simulink model "AGV_Simulation_Follow"  (R2022a)
settings: Solver=VariableStepAuto  StartTime=0.0  StopTime=200  RelTol=1e-3  EnableMultiTasking=on
undefined symbols (not defined in the file or in its folder): Final_path, gray, lastx, lasty, Rec, SDTV, start
libraries: vrlib x6, visionconversions x2, robotalgslib x1, visionanalysis x1, visiontextngfix x1
settings Model: Creator=Carlos  LastModifiedBy=a22adhpa
settings SolverCC: AlgebraicLoopSolver=TrustRegion
settings DataIOCC: LimitDataPoints=on  MaxDataPoints=10000
settings OptimizationCC: LifeSpan=inf
settings DebuggingCC: UnconnectedInputMsg=warning  UnconnectedOutputMsg=warning  UnconnectedLineMsg=warning  AllowSymbolicDim=off  SFUnexpectedBacktrackingDiag=warning  SFNoUnconditionalDefaultTransitionDiag=warning  SFExecutionAtInitializationDiag=none  SFMachineParentedDataDiag=warning  UnderSpecifiedDimensionMsg=warning  ArithmeticOperatorsInVariantConditions=warning
settings SFSimCC: SimUseLocalCustomCode=off  CustomCodeUndefinedFunction=UseInterfaceOnly
settings RTWCC: RTWUseLocalCustomCode=off
settings CodeAppCC: StateflowObjectComments=on
settings GRTTargetCC: TargetLangStandard=C89/C90 (ANSI)
settings ConfigComp: CovMetricSettings=dw  CovSaveCumulativeToWorkspaceVar=on  CovSaveSingleToWorkspaceVar=on  CovExternalEMLEnable=off  CovSFcnEnable=off
settings SimscapeCC: SimscapeLogType=all  SimscapeLogSimulationStatistics=on  SimscapeLogDataHistory=10000

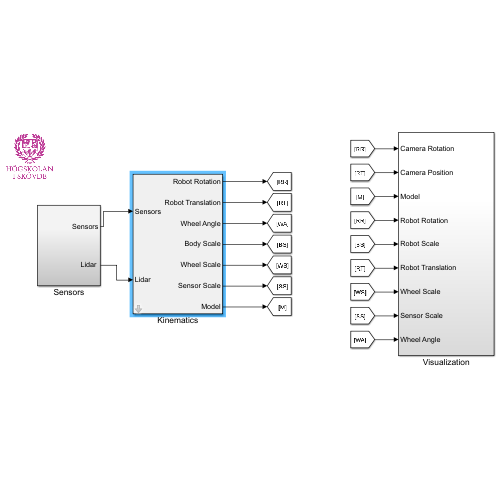
[thumbnail: Simulink's stored preview of the top-level diagram]
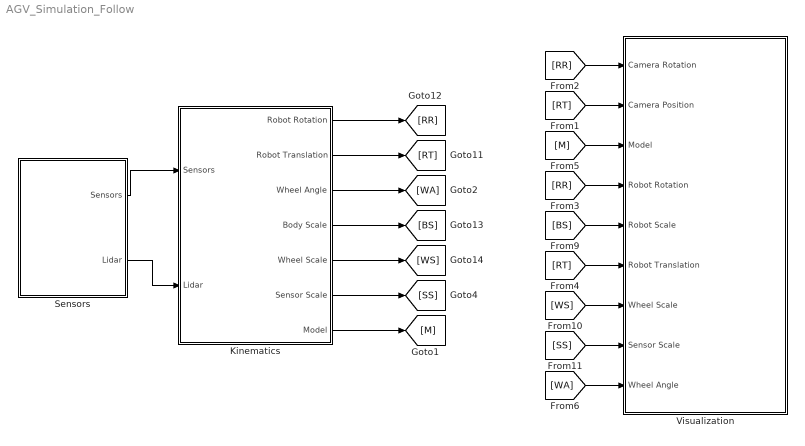
== system AGV_Simulation_Follow ==
  Kinematics : Subsystem  mask(Simulation Parameters){Op=Differential Drive, Kim=Inverse, DimR=[0.6, 0.5, 0.15], DimW=[0.18, 0.12], InitPos=start, InitRot=0, Dim=[1.00,1.00,0.15;1.40,0.80,0.15;1.40,0.8,0.15;1.2,0.8,0.15]}
      mask prompts: Op "Robot Models:"; Kim "Kinematics:"; DimR "Robot Dimensions (m)"; DimW "Wheel Dimensions (m)"; InitPos "Initial Position (m)"; InitRot "Initial Rotation (rad)"; Dim "Dimensions (m)"
      mask help: Define the dimensions of the robot [Length, Width, Thickness] and of the wheels [Radius, Thickness].
      mask TypeOptions Op: Differential Drive | Tricycle Drive | Ackermann Steering | Swedish Model
      mask TypeOptions Kim: Forward | Inverse
      mask DialogControl Control Prompt: Select the robot and kinematics used for the algorithms.
      mask DialogControl DescTextVar_copy Prompt: Define the dimensions of the robot [Length, Width, Thickness] and of the wheels [Radius, Thickness]:
      mask DialogControl DescTextVar Prompt: Set the initial position [X Z] and rotation [Angle] of the robot:
  Sensors : Subsystem
  Visualization : Subsystem
  wires:
  Kinematics/2(Robot Translation) -> [RT]
  Kinematics/1(Robot Rotation) -> [RR]
  Kinematics/4(Body Scale) -> [BS]
  Kinematics/5(Wheel Scale) -> [WS]
  Kinematics/6(Sensor Scale) -> [SS]
  Kinematics/7(Model) -> [M]
  [RR] -> Visualization/1(Camera Rotation)
  [RT] -> Visualization/2(Camera Position)
  [M] -> Visualization/3(Model)
  [RR] -> Visualization/4(Robot Rotation)
  [BS] -> Visualization/5(Robot Scale)
  [WS] -> Visualization/7(Wheel Scale)
  [SS] -> Visualization/8(Sensor Scale)
  Kinematics/3(Wheel Angle) -> [WA]
  [WA] -> Visualization/9(Wheel Angle)
  [RT] -> Visualization/6(Robot Translation)
  Sensors/1(Sensors) -> Kinematics/1(Sensors)
  Sensors/2("Lidar ") -> Kinematics/2(Lidar)

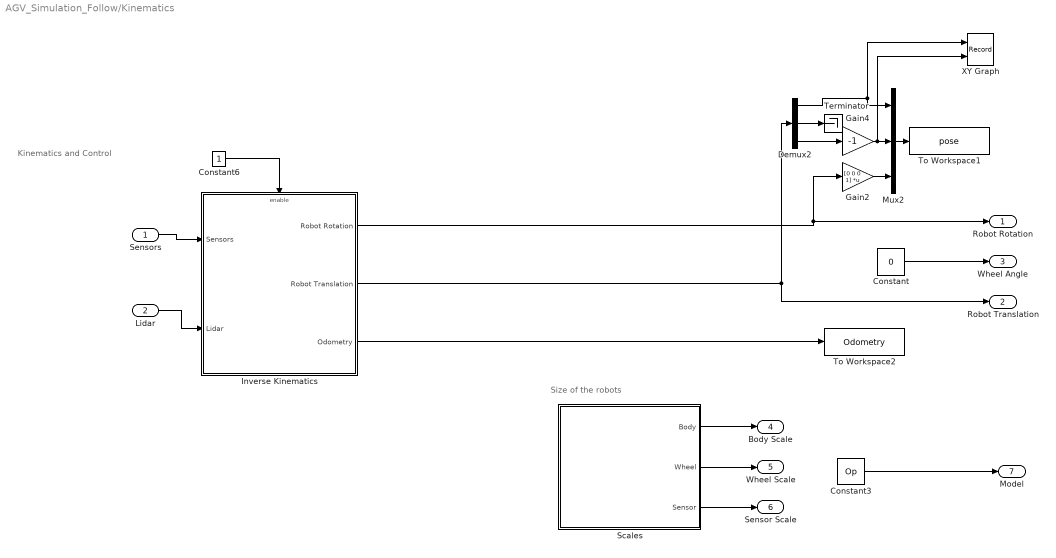
== system AGV_Simulation_Follow/Kinematics ==
  note: Size of the robots
  note: Kinematics and Control
  Sensors : Inport
  Lidar : Inport  Port=2
  Constant : Constant  Value=0
  Constant3 : Constant  Value=Op
  Constant6 : Constant
  Demux2 : Demux  Outputs=3
  Gain2 : Gain  Gain=[0 0 0 1]  Multiplication=Matrix(K*u)
  Gain4 : Gain  Gain=-1
  Inverse Kinematics : Subsystem
  Mux2 : Mux  Inputs=3
  Scales : Subsystem
  Terminator : Terminator
  To Workspace1 : ToWorkspace  VariableName=pose  SaveFormat=Timeseries  SampleTime=1
  To Workspace2 : ToWorkspace  VariableName=Odometry  SaveFormat=Timeseries  SampleTime=1
  XY Graph : Record  FileSettingsInternal="{\"entries\":[{\"content\":{\"excelSettings\":{\"content\":{},\"type\":\"Streamout.ExcelSettings\"}},\"type\":\"Streamout.FileSettingStorage\",\"uuid\":\"f8be6537-237c-46b6-b0f9-78c47728e387\"}],\"packageUris\":[\"http://schema.mathworks.com/mf0/streamout_blocks/R2020a\"],\"version\":\"1.0\"}"  Layout=[1 1]  SignalsInternal="{\"entries\":[{\"content\":{\"signals\":[{\"content\":{\"blockPath\":[\"AGV_Simulation_Follow/Kinematics/XY Graph\"],\"channel\":[],\"dimensions\":[1],\"domain\":\"AGV_Simulation_Follow/Kinematics/XY Graph\",\"lineColor\":\"#a2142f\",\"plots\":[1],\"port\":1,\"sid\":[\"\"],\"signalID\":4787,\"signalName\":\"Demux2:1\"},\"type\":\"RecordBlkView.Signal\",\"uuid\":\"16ab8450-91a6-44a9-b9b9-14d5707b15d7\"},{\"content\":{\"blockPath\":[\"AGV_Simulation_Follow/Kinematics/XY Graph\"],\"channel\":[],\"dimensions\":[1],\"domain\":\"AGV_Simulation_Follow/Kinematics/XY Graph\",\"lineColor\":\"#139fff\",\"plots\":[1],\"port\":2,\"sid\":[\"\"],\"signalID\":4791,\"signalName\":\"Gain4\"},\"type\":\"RecordBlkView.Signal\",\"uuid\":\"b7748771-608b-4166-b0c9-3eeaa203ac76\"}]},\"type\":\"RecordBlkView.InputSignals\",\"uuid\":\"e4230418-6337-4a24-a4ca-903df54e3671\"}],\"packageUris\":[\"http://schema.mathworks.com/mf0/streamout_blocks/R2020a\"],\"version\":\"1.0\"}"  VisualizationBindings="{\"xyplotplugin\":{\"info\":[{\"series\":[{\"bindingParametersList\":[{\"parameter\":\"X-Axis\",\"signalID\":4787,\"signalName\":\"Demux2:1\"},{\"parameter\":\"Y-Axis\",\"signalID\":4791,\"signalName\":\"Gain4\"}],\"seriesID\":48962}],\"subplotID\":1}]}}"  CompatibilityTag=XY  st=1
  Robot Rotation : Outport
  Robot Translation : Outport  Port=2
  Wheel Angle : Outport  Port=3
  Body Scale : Outport  Port=4
  Wheel Scale : Outport  Port=5
  Sensor Scale : Outport  Port=6
  Model : Outport  Port=7
  wires:
  Scales/1(Body) -> Body Scale/1
  Scales/3(Sensor) -> Sensor Scale/1
  Scales/2(Wheel) -> Wheel Scale/1
  Sensors/1 -> Inverse Kinematics/1(Sensors)
  Constant3/1 -> Model/1
  Inverse Kinematics/2(Robot Translation) -> Robot Translation/1, Demux2/1
  Constant6/1 -> Inverse Kinematics/Enable
  Gain4/1 -> XY Graph/2, Mux2/2
  Demux2/1 -> Mux2/1, XY Graph/1
  Inverse Kinematics/1(Robot Rotation) -> Gain2/1, Robot Rotation/1
  Mux2/1 -> To Workspace1/1
  Demux2/3 -> Gain4/1
  Gain2/1 -> Mux2/3
  Constant/1 -> Wheel Angle/1
  Inverse Kinematics/3(Odometry) -> To Workspace2/1
  Lidar/1 -> Inverse Kinematics/2(Lidar)
  Demux2/2 -> Terminator/1

== system AGV_Simulation_Follow/Sensors ==
  Mux : Mux
  To Workspace1 : ToWorkspace  VariableName=Rang  SaveFormat=Timeseries  SampleTime=1
      settings: Save2DSignal=2-D array (concatenate along first dimension)
  VR Source : vrlib/VR Source  InstantiateOnLoad=on  SampleTime=0.1  ViewEnable=on  RemoteChange=off  RemoteView=off  FieldsRead=Diff_SensorF.isActive.1.1.1.logical#Diff_SensorR.isActive.1.1.1.logical#Diff_SensorL.isActive.1.1.1.logical#Diff_SensorB.isActive.1.1.1.logical#SLAM_Sensor.pickedRange.240.1.1.double  WorldFileName=Scenario.x3d  WorldDescription=Template Robot Simulation  AutoView=off  VideoDimensions=[]  AllowVariableSize=off
      settings: SourceProductBaseCode=SL
  Sensors : Outport
  "Lidar " : Outport  Port=2
  wires:
  Mux/1 -> Sensors/1
  VR Source/1 -> Mux/1
  VR Source/2 -> Mux/2
  VR Source/3 -> Mux/3
  VR Source/4 -> Mux/4
  VR Source/5 -> To Workspace1/1, "Lidar "/1

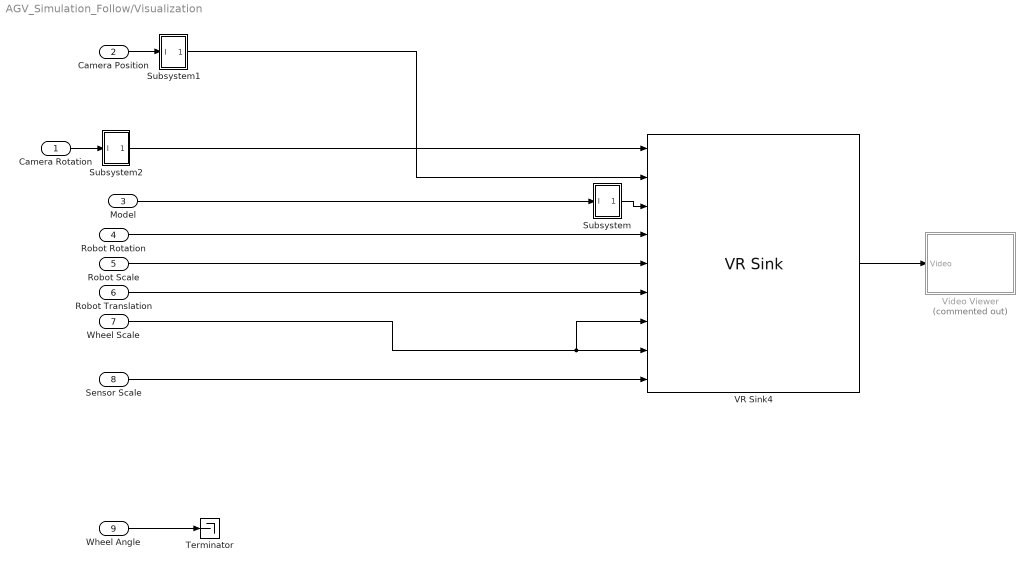
== system AGV_Simulation_Follow/Visualization ==
  Camera Rotation : Inport
  Camera Position : Inport  Port=2
  Model : Inport  Port=3
  Robot Rotation : Inport  Port=4
  Robot Scale : Inport  Port=5
  Robot Translation : Inport  Port=6
  Wheel Scale : Inport  Port=7
  Sensor Scale : Inport  Port=8
  Wheel Angle : Inport  Port=9
  Subsystem : Subsystem
  Subsystem1 : Subsystem
  Subsystem2 : Subsystem
  Terminator : Terminator
  VR Sink4 : vrlib/VR Sink  InstantiateOnLoad=on  SampleTime=0.1  ViewEnable=on  RemoteChange=off  RemoteView=off  FieldsWritten=Sensor_Camera.orientation.4.1.1.double#Sensor_Camera.position.3.1.1.double#Kinematic_Models.whichChoice.1.1.1.double#Differential_Drive.rotation.4.1.1.double#Differential_Drive.scale.3.1.1.double#Differential_Drive.translation.3.1.1.double#Right_Wheel.scale.3.1.1.double#Left_Wheel.scale.3.1.1.double#Sensors_Diff.scale.3.1.1.double  WorldFileName=Scenario.x3d  WorldDescription=Template Robot Simulation  AutoView=off  VideoDimensions=[480 640]  AllowVariableSize=off  FigureProperties="{'Position', 'Name', 'Viewpoint', 'CameraBound', 'CameraDirection', 'CameraPosition', 'CameraUpVector', 'ZoomFactor', 'Antialiasing', 'Headlight', 'Lighting', 'NavPanel', 'Sound', 'StatusBar', 'Stereo3D', 'Stereo3DCameraOffset', 'Stereo3DHIT', 'ToolBar', 'Textures', 'Transparency', 'Triad', 'Wireframe', 'NavZones', 'NavMode', 'NavSpeed', 'CaptureFileFormat', 'CaptureFileName', 'Record2DCompressMethod', 'Record2DCompressQuality', 'Record2D', 'Record2DFileName', 'Record2DFPS'; [5.8600000000000000e+02   6.0000000000000000e+01   6.2400000000000000e+02   4.0000000000000000e+02], 'Dynamics Visualization', 'Top', 'on', [0.0000000000000000e+00   0.0000000000000000e+00  -1.0000000000000000e+00], [0.0000000000000000e+00   0.0000000000000000e+00   0.0000000000000000e+00], [0.0000000000000000e+00   1.0000000000000000e+00   0.0000000000000000e+00], [1.0000000000000000e+00], 'on', 'on', 'on', 'none', 'on', 'off', 'off', [1.0000000149011612e-01], [0.0000000000000000e+00], 'off', 'on', 'on', 'none', 'off', 'off', 'fly', 'normal', 'tif', '%f_anim_%n.tif', 'auto', [7.5000000000000000e+01], 'off', '***video***', 'auto'}"
  Video Viewer : Subsystem  Commented=on
  wires:
  Wheel Angle/1 -> Terminator/1
  Camera Rotation/1 -> Subsystem2/1(I)
  Camera Position/1 -> Subsystem1/1(I)
  Model/1 -> Subsystem/1(I)
  VR Sink4/1 -> Video Viewer/1(Video)
  Sensor Scale/1 -> VR Sink4/9
  Wheel Scale/1 -> VR Sink4/7, VR Sink4/8
  Robot Translation/1 -> VR Sink4/6
  Robot Scale/1 -> VR Sink4/5
  Robot Rotation/1 -> VR Sink4/4
  Subsystem1/1(O) -> VR Sink4/2
  Subsystem/1(O) -> VR Sink4/3
  Subsystem2/1(O) -> VR Sink4/1

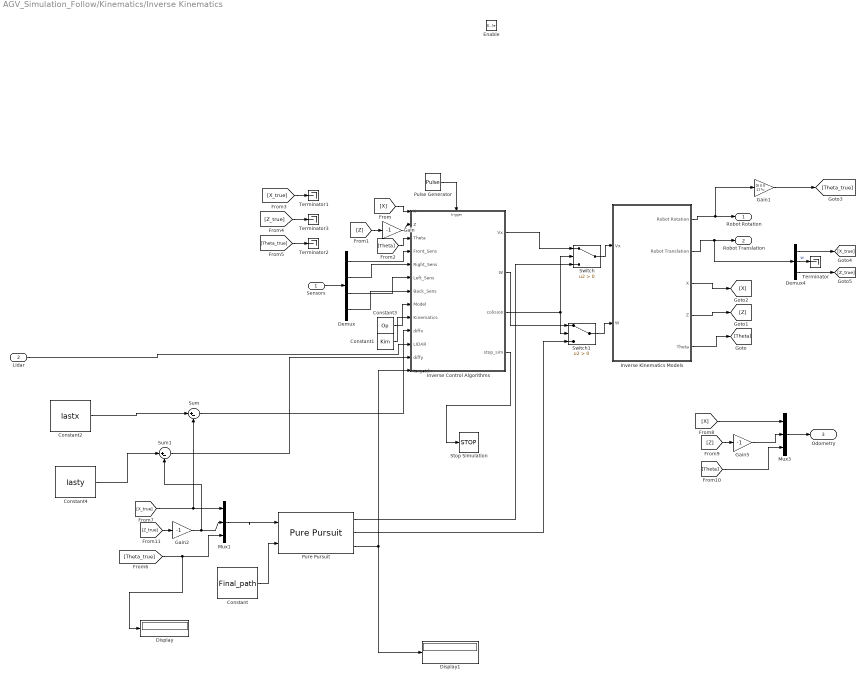
== system AGV_Simulation_Follow/Kinematics/Inverse Kinematics ==
  Sensors : Inport
  Lidar : Inport  Port=2
  Enable : EnablePort
  Constant : Constant  Value=Final_path
  Constant1 : Constant  Value=Kim
  Constant2 : Constant  Value=lastx
  Constant3 : Constant  Value=Op
  Constant4 : Constant  Value=lasty
  Demux : Demux
  Demux4 : Demux  Outputs=3
  Display : Display
  Display1 : Display
  Gain : Gain  Gain=-1
  Gain1 : Gain  Gain=[0 0 0 1]  Multiplication=Matrix(K*u)
  Gain2 : Gain  Gain=-1
  Gain5 : Gain  Gain=-1
  Inverse Control Algorithms : Stateflow chart  TreatAsAtomicUnit=on
  Inverse Kinematics Models : Subsystem
  Mux1 : Mux  Inputs=3
  Mux3 : Mux  Inputs=3
  Pulse Generator : DiscretePulseGenerator  PulseType=Time based  Period=0.02  PulseWidth=50
  Pure Pursuit : robotalgslib/Pure Pursuit  DesiredLinearVelocity=0.75  MaxAngularVelocity=2.0  LookaheadDistance=1.0  TargetDirPort=on  SimulateUsing=Code generation
  Stop Simulation : Stop
  Sum : Sum  Inputs=|+-
  Sum1 : Sum  Inputs=|+-
  Switch : Switch  Criteria=u2 > Threshold  SaturateOnIntegerOverflow=off  InputSameDT=off
  Switch1 : Switch  Criteria=u2 > Threshold  SaturateOnIntegerOverflow=off  InputSameDT=off
  Terminator{,1..3} (4 alike) : Terminator
  Robot Rotation : Outport
  Robot Translation : Outport  Port=2
  Odometry : Outport  Port=3
  wires:
  [Theta] -> Inverse Control Algorithms/3(Theta)
  Inverse Kinematics Models/3(X) -> [X]
  Inverse Kinematics Models/5(Theta) -> [Theta]
  [Z] -> Gain/1
  Pulse Generator/1 -> Inverse Control Algorithms/Trigger
  Constant3/1 -> Inverse Control Algorithms/8(Model)
  Inverse Control Algorithms/1(Vx) -> Switch/1
  Inverse Kinematics Models/4(Z) -> [Z]
  [X] -> Inverse Control Algorithms/1(X)
  Inverse Control Algorithms/2(W) -> Switch1/1
  Constant1/1 -> Inverse Control Algorithms/9(Kinematics)
  Demux/2 -> Inverse Control Algorithms/5(Right_Sens)
  Demux/3 -> Inverse Control Algorithms/6(Left_Sens)
  Demux/1 -> Inverse Control Algorithms/4(Front_Sens)
  Sensors/1 -> Demux/1
  Demux/4 -> Inverse Control Algorithms/7(Back_Sens)
  Gain/1 -> Inverse Control Algorithms/2(Z)
  Mux3/1 -> Odometry/1
  [X] -> Mux3/1
  [Theta] -> Mux3/3
  [Z] -> Gain5/1
  Gain5/1 -> Mux3/2
  Inverse Kinematics Models/2(Robot Translation) -> Demux4/1, Robot Translation/1
  Inverse Kinematics Models/1(Robot Rotation) -> Gain1/1, Robot Rotation/1
  Demux4/2 -> Terminator/1  "w"
  Demux4/3 -> [Z_true]
  Demux4/1 -> [X_true]
  Gain1/1 -> [Theta_true]
  [Theta_true] -> Terminator2/1
  [Z_true] -> Terminator3/1
  [X_true] -> Terminator1/1
  [Z_true] -> Gain2/1
  [Theta_true] -> Display/1, Mux1/3
  Mux1/1 -> Pure Pursuit/1
  [X_true] -> Sum/2, Mux1/1
  Gain2/1 -> Sum1/2, Mux1/2
  Constant/1 -> Pure Pursuit/2
  Switch/1 -> Inverse Kinematics Models/1(Vx)
  Switch1/1 -> Inverse Kinematics Models/2(W)
  Inverse Control Algorithms/3(colision) -> Switch/2, Switch1/2
  Pure Pursuit/3 -> Display1/1, Inverse Control Algorithms/13(targetdir)
  Pure Pursuit/1 -> Switch/3
  Pure Pursuit/2 -> Switch1/3
  Lidar/1 -> Inverse Control Algorithms/11(LIDAR)
  Constant2/1 -> Sum/1
  Sum/1 -> Inverse Control Algorithms/10(diffx)
  Constant4/1 -> Sum1/1
  Sum1/1 -> Inverse Control Algorithms/12(diffy)
  Inverse Control Algorithms/4(stop_sim) -> Stop Simulation/1

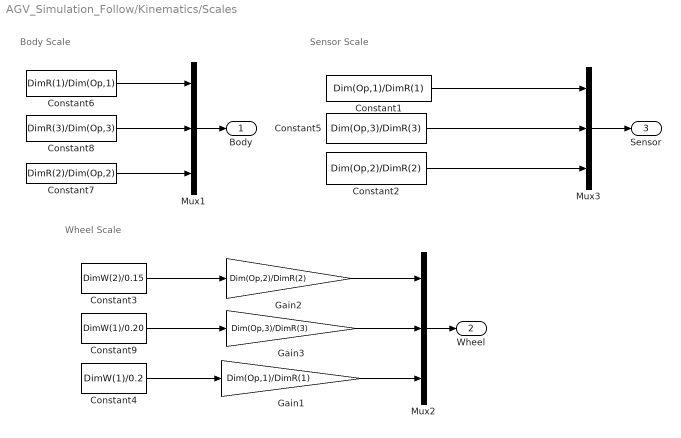
== system AGV_Simulation_Follow/Kinematics/Scales ==
  note: Body Scale
  note: Wheel Scale
  note: Sensor Scale
  Constant1 : Constant  Value=Dim(Op,1)/DimR(1)
  Constant2 : Constant  Value=Dim(Op,2)/DimR(2)
  Constant3 : Constant  Value=DimW(2)/0.15
  Constant4 : Constant  Value=DimW(1)/0.2
  Constant5 : Constant  Value=Dim(Op,3)/DimR(3)
  Constant6 : Constant  Value=DimR(1)/Dim(Op,1)
  Constant7 : Constant  Value=DimR(2)/Dim(Op,2)
  Constant8 : Constant  Value=DimR(3)/Dim(Op,3)
  Constant9 : Constant  Value=DimW(1)/0.20
  Gain1 : Gain  Gain=Dim(Op,1)/DimR(1)
  Gain2 : Gain  Gain=Dim(Op,2)/DimR(2)
  Gain3 : Gain  Gain=Dim(Op,3)/DimR(3)
  Mux1 : Mux  Inputs=3
  Mux2 : Mux  Inputs=3
  Mux3 : Mux  Inputs=3
  Body : Outport
  Wheel : Outport  Port=2
  Sensor : Outport  Port=3
  wires:
  Mux3/1 -> Sensor/1
  Mux2/1 -> Wheel/1
  Mux1/1 -> Body/1
  Constant2/1 -> Mux3/3
  Constant5/1 -> Mux3/2
  Constant1/1 -> Mux3/1
  Gain2/1 -> Mux2/1
  Constant3/1 -> Gain2/1
  Constant7/1 -> Mux1/3
  Constant6/1 -> Mux1/1
  Constant8/1 -> Mux1/2
  Constant4/1 -> Gain1/1
  Constant9/1 -> Gain3/1
  Gain3/1 -> Mux2/2
  Gain1/1 -> Mux2/3

== system AGV_Simulation_Follow/Visualization/Subsystem ==
  I : Inport
  Constant3 : Constant
  Subtract : Sum  Inputs=+-
  O : Outport
  wires:
  Subtract/1 -> O/1
  Constant3/1 -> Subtract/2
  I/1 -> Subtract/1

== system AGV_Simulation_Follow/Visualization/Subsystem1 ==
  I : Inport
  Constant3 : Constant  Value=[0 0.7 0]
  Subtract : Sum
  O : Outport
  wires:
  Subtract/1 -> O/1
  Constant3/1 -> Subtract/2
  I/1 -> Subtract/1

== system AGV_Simulation_Follow/Visualization/Subsystem2 ==
  I : Inport
  Constant3 : Constant  Value=[0 1 0 -pi/2]
  Subsystem3 : Subsystem  Commented=on
  Subtract : Sum
  O : Outport
  wires:
  Subtract/1 -> O/1
  Constant3/1 -> Subtract/2
  I/1 -> Subtract/1

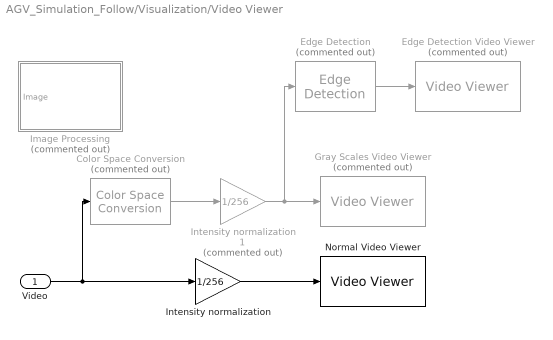
== system AGV_Simulation_Follow/Visualization/Video Viewer ==
  Video : Inport
  Color Space Conversion : visionconversions/Color Space  Conversion  Commented=on  conversion=Obsolete  conversionActive=R'G'B' to intensity  wp_str=D65  rec=Rec. 601 (SDTV)  sys=1125/60/2:1  imagePorts=One multidimensional signal
  Edge Detection : visionanalysis/Edge Detection  Commented=on  method=Sobel  outputType=Binary image  userDefinedThreshold=off  thresholdSource=Input port  threshold=20  thresholdTuning=2  edgeThinning=off  threshold_canny=[0.25 0.60]  autoPercent=70  sigma=1  roundingMode=Floor  overflowMode=off  prodOutputMode=Binary point scaling  prodOutputWordLength=32  prodOutputFracLength=8
      settings: SourceProductBaseCode=VP
  Edge Detection Video Viewer : VideoViewer  Commented=on  colormapValue=gray(256)  FigPos=[393 765 681 657]  trueSizedOnce=on
  Gray Scales Video Viewer : VideoViewer  Commented=on  colormapValue=gray(256)  FigPos=[685 765 681 657]  trueSizedOnce=on
  Image Processing : Subsystem  Commented=on
  Intensity normalization : Gain  Gain=1/256  OutDataTypeStr=double
  Intensity normalization1 : Gain  Commented=on  Gain=1/256  OutDataTypeStr=double
  Normal Video Viewer : VideoViewer  colormapValue=gray(256)  FigPos=[1903.4 908.4 855.2 630.4]  trueSizedOnce=on
  wires:
  Intensity normalization/1 -> Normal Video Viewer/1
  Video/1 -> Intensity normalization/1, Color Space Conversion/1
  Color Space Conversion/1 -> Intensity normalization1/1
  Intensity normalization1/1 -> Edge Detection/1, Gray Scales Video Viewer/1
  Edge Detection/1 -> Edge Detection Video Viewer/1

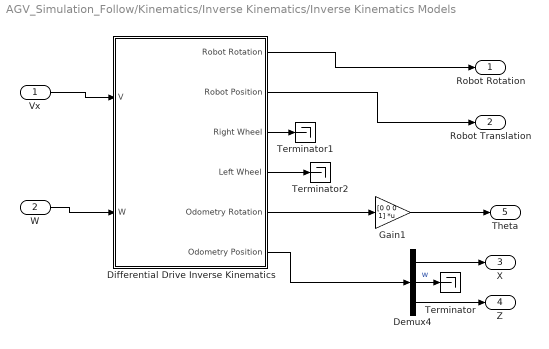
== system AGV_Simulation_Follow/Kinematics/Inverse Kinematics/Inverse Kinematics Models ==
  Vx : Inport
  W : Inport  Port=2
  Demux4 : Demux  Outputs=3
  Differential Drive Inverse Kinematics : Subsystem
  Gain1 : Gain  Gain=[0 0 0 1]  Multiplication=Matrix(K*u)
  Terminator : Terminator
  Terminator1 : Terminator
  Terminator2 : Terminator
  Robot Rotation : Outport
  Robot Translation : Outport  Port=2
  X : Outport  Port=3
  Z : Outport  Port=4
  Theta : Outport  Port=5
  wires:
  Differential Drive Inverse Kinematics/2(Robot Position) -> Robot Translation/1
  Demux4/1 -> X/1
  Demux4/3 -> Z/1
  Differential Drive Inverse Kinematics/1(Robot Rotation) -> Robot Rotation/1
  Vx/1 -> Differential Drive Inverse Kinematics/1(V)
  W/1 -> Differential Drive Inverse Kinematics/2(W)
  Gain1/1 -> Theta/1
  Demux4/2 -> Terminator/1  "w"
  Differential Drive Inverse Kinematics/3(Right Wheel) -> Terminator1/1
  Differential Drive Inverse Kinematics/4(Left Wheel) -> Terminator2/1
  Differential Drive Inverse Kinematics/6(Odometry Position) -> Demux4/1
  Differential Drive Inverse Kinematics/5(Odometry Rotation) -> Gain1/1

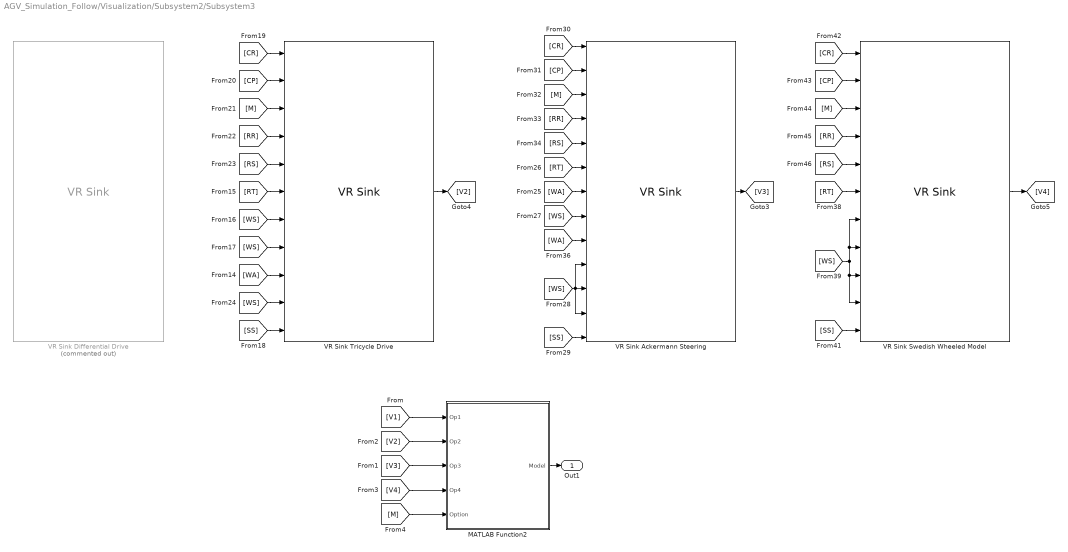
== system AGV_Simulation_Follow/Visualization/Subsystem2/Subsystem3 ==
  MATLAB Function2 : MATLAB Function  TreatAsAtomicUnit=on
  VR Sink Ackermann Steering : vrlib/VR Sink  InstantiateOnLoad=on  SampleTime=0.1  ViewEnable=on  RemoteChange=off  RemoteView=off  FieldsWritten=Sensor_Camera.orientation.4.1.1.double#Sensor_Camera.position.3.1.1.double#Kinematic_Models.whichChoice.1.1.1.double#Ackerman_Steering.rotation.4.1.1.double#Ackerman_Steering.scale.3.1.1.double#Ackerman_Steering.translation.3.1.1.double#Front_Right_Wheel.rotation.4.1.1.double#Front_Right_Wheel.scale.3.1.1.double#Front_Left_Wheel.rotation.4.1.1.double#Front_Left_Wheel.scale.3.1.1.double#Rear_Right_Wheel.scale.3.1.1.double#Rear_Left_Wheel.scale.3.1.1.double#Sensors_Ack.scale.3.1.1.double  WorldFileName=Scenario.WRL  WorldDescription=Dynamics Visualization  AutoView=off  VideoDimensions=[400 624]  AllowVariableSize=off
  VR Sink Differential Drive : vrlib/VR Sink  Commented=on  InstantiateOnLoad=on  SampleTime=0.1  ViewEnable=on  RemoteChange=off  RemoteView=off  FieldsWritten=Sensor_Camera.orientation.4.1.1.double#Sensor_Camera.position.3.1.1.double#Kinematic_Models.whichChoice.1.1.1.double#Differential_Drive.rotation.4.1.1.double#Differential_Drive.scale.3.1.1.double#Differential_Drive.translation.3.1.1.double#Left_Wheel.scale.3.1.1.double#Right_Wheel.scale.3.1.1.double#Sensors_Diff.scale.3.1.1.double  WorldFileName=Scenario.WRL  WorldDescription=Dynamics Visualization  AutoView=on  VideoDimensions=[400 624]  AllowVariableSize=off  FigureProperties="{'Position', 'Name', 'Viewpoint', 'CameraBound', 'CameraDirection', 'CameraPosition', 'CameraUpVector', 'ZoomFactor', 'Antialiasing', 'Headlight', 'Lighting', 'NavPanel', 'Sound', 'StatusBar', 'Stereo3D', 'Stereo3DCameraOffset', 'Stereo3DHIT', 'ToolBar', 'Textures', 'Transparency', 'Triad', 'Wireframe', 'NavZones', 'NavMode', 'NavSpeed', 'CaptureFileFormat', 'CaptureFileName', 'Record2DCompressMethod', 'Record2DCompressQuality', 'Record2D', 'Record2DFileName', 'Record2DFPS'; [5.8600000000000000e+02   6.0000000000000000e+01   6.2400000000000000e+02   4.0000000000000000e+02], 'Dynamics Visualization', 'Sensor Camera', 'on', [0.0000000000000000e+00   0.0000000000000000e+00  -1.0000000000000000e+00], [0.0000000000000000e+00   0.0000000000000000e+00   0.0000000000000000e+00], [0.0000000000000000e+00   1.0000000000000000e+00   0.0000000000000000e+00], [1.0000000000000000e+00], 'on', 'on', 'on', 'none', 'on', 'off', 'off', [1.0000000149011612e-01], [0.0000000000000000e+00], 'off', 'on', 'on', 'none', 'off', 'off', 'fly', 'normal', 'tif', '%f_anim_%n.tif', 'auto', [7.5000000000000000e+01], 'off', '***video***', 'auto'}"
  VR Sink Swedish Wheeled Model : vrlib/VR Sink  InstantiateOnLoad=on  SampleTime=0.1  ViewEnable=on  RemoteChange=off  RemoteView=off  FieldsWritten=Sensor_Camera.orientation.4.1.1.double#Sensor_Camera.position.3.1.1.double#Kinematic_Models.whichChoice.1.1.1.double#Swedish_Wheeled_Model.rotation.4.1.1.double#Swedish_Wheeled_Model.scale.3.1.1.double#Swedish_Wheeled_Model.translation.3.1.1.double#Front_Right.scale.3.1.1.double#Front_Left.scale.3.1.1.double#Rear_Right.scale.3.1.1.double#Rear_Left.scale.3.1.1.double#Sensors3.scale.3.1.1.double  WorldFileName=Scenario.WRL  WorldDescription=Dynamics Visualization  AutoView=off  VideoDimensions=[400 624]  AllowVariableSize=off
  VR Sink Tricycle Drive : vrlib/VR Sink  InstantiateOnLoad=on  SampleTime=0.1  ViewEnable=on  RemoteChange=off  RemoteView=off  FieldsWritten=Sensor_Camera.orientation.4.1.1.double#Sensor_Camera.position.3.1.1.double#Kinematic_Models.whichChoice.1.1.1.double#Tricycle_Drive.rotation.4.1.1.double#Tricycle_Drive.scale.3.1.1.double#Tricycle_Drive.translation.3.1.1.double#Left_Wheel_Tri.scale.3.1.1.double#Right_Wheel_Tri.scale.3.1.1.double#Front_Wheel.rotation.4.1.1.double#Front_Wheel.scale.3.1.1.double#Sensors_Tri.scale.3.1.1.double  WorldFileName=Scenario.WRL  WorldDescription=Dynamics Visualization  AutoView=on  VideoDimensions=[400 624]  AllowVariableSize=off
  Out1 : Outport
  wires:
  [V1] -> MATLAB Function2/1(Op1)
  [CP] -> VR Sink Swedish Wheeled Model/2
  [WS] -> VR Sink Swedish Wheeled Model/7, VR Sink Swedish Wheeled Model/8, VR Sink Swedish Wheeled Model/10, VR Sink Swedish Wheeled Model/9
  [RR] -> VR Sink Tricycle Drive/4
  VR Sink Tricycle Drive/1 -> [V2]
  [CP] -> VR Sink Tricycle Drive/2
  [CR] -> VR Sink Ackermann Steering/1
  [SS] -> VR Sink Tricycle Drive/11
  [WA] -> VR Sink Ackermann Steering/9
  [CR] -> VR Sink Swedish Wheeled Model/1
  [WS] -> VR Sink Ackermann Steering/12, VR Sink Ackermann Steering/10, VR Sink Ackermann Steering/11
  [WS] -> VR Sink Tricycle Drive/7
  [WS] -> VR Sink Tricycle Drive/8
  [M] -> VR Sink Ackermann Steering/3
  [RS] -> VR Sink Swedish Wheeled Model/5
  [RT] -> VR Sink Swedish Wheeled Model/6
  [SS] -> VR Sink Ackermann Steering/13
  MATLAB Function2/1(Model) -> Out1/1
  [RT] -> VR Sink Tricycle Drive/6
  [SS] -> VR Sink Swedish Wheeled Model/11
  VR Sink Swedish Wheeled Model/1 -> [V4]
  [V3] -> MATLAB Function2/3(Op3)
  [V4] -> MATLAB Function2/4(Op4)
  [V2] -> MATLAB Function2/2(Op2)
  [WA] -> VR Sink Ackermann Steering/7
  [WS] -> VR Sink Ackermann Steering/8
  [M] -> VR Sink Tricycle Drive/3
  [RS] -> VR Sink Tricycle Drive/5
  [WA] -> VR Sink Tricycle Drive/9
  [WS] -> VR Sink Tricycle Drive/10
  VR Sink Ackermann Steering/1 -> [V3]
  [CP] -> VR Sink Ackermann Steering/2
  [RR] -> VR Sink Swedish Wheeled Model/4
  [RS] -> VR Sink Ackermann Steering/5
  [M] -> VR Sink Swedish Wheeled Model/3
  [M] -> MATLAB Function2/5(Option)
  [RR] -> VR Sink Ackermann Steering/4
  [RT] -> VR Sink Ackermann Steering/6
  [CR] -> VR Sink Tricycle Drive/1

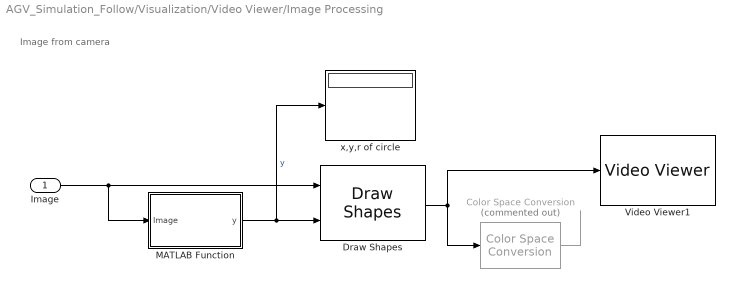
== system AGV_Simulation_Follow/Visualization/Video Viewer/Image Processing ==
  note: Image from camera
  Image : Inport
  Color Space Conversion : visionconversions/Color Space  Conversion  Commented=on  conversion=Obsolete  conversionActive=R'G'B' to intensity  wp_str=D65  rec=Rec. 601 (SDTV)  sys=1125/60/2:1  imagePorts=One multidimensional signal
  Draw Shapes : visiontextngfix/Draw Shapes  shape=Circles  fill=off  lineWidth=2  fillClrSource=Specify via dialog  display=White  intensity=200  color=[200 255 100]  opacity=0.6  viewport=Entire image  antialiasing=off  inType=Obsolete  imagePorts=One multidimensional signal  roundingMode=Floor  overflowMode=off  memoryMode=Specify word length  memoryWordLength=16  prodOutputMode=Binary point scaling  prodOutputWordLength=32  prodOutputFracLength=14  memoryFracLength=15
  MATLAB Function : MATLAB Function  TreatAsAtomicUnit=on
  Video Viewer1 : VideoViewer  FigPos=[23 808 1370 668]
  x,y,r of circle : Display
  wires:
  MATLAB Function/1(y) -> x,y,r of circle/1, Draw Shapes/2  "y"
  Image/1 -> MATLAB Function/1(Image), Draw Shapes/1
  Draw Shapes/1 -> Video Viewer1/1, Color Space Conversion/1
  Color Space Conversion/1 -> ?

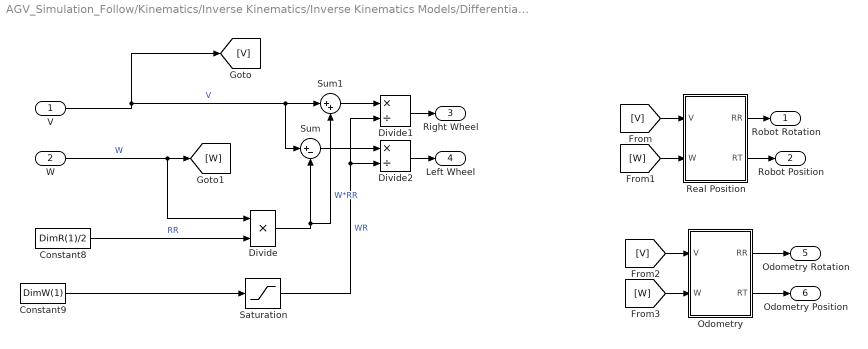
== system AGV_Simulation_Follow/Kinematics/Inverse Kinematics/Inverse Kinematics Models/Differential Drive Inverse Kinematics ==
  V : Inport
  W : Inport  Port=2
  Constant8 : Constant  Value=DimR(1)/2
  Constant9 : Constant  Value=DimW(1)
  Divide : Product  Inputs=**
  Divide1 : Product  Inputs=*/
  Divide2 : Product  Inputs=*/
  Odometry : Subsystem
  Real Position : Subsystem
  Saturation : Saturate  UpperLimit=10  LowerLimit=0.01
  Sum : Sum  Inputs=|+-
  Sum1 : Sum  Inputs=|++
  Robot Rotation : Outport
  Robot Position : Outport  Port=2
  Right Wheel : Outport  Port=3
  Left Wheel : Outport  Port=4
  Odometry Rotation : Outport  Port=5
  Odometry Position : Outport  Port=6
  wires:
  V/1 -> [V], Sum/1, Sum1/1  "V"
  W/1 -> Divide/1, [W]  "W"
  Constant8/1 -> Divide/2  "RR"
  Constant9/1 -> Saturation/1
  [V] -> Real Position/1(V)
  [W] -> Real Position/2(W)
  Real Position/1(RR) -> Robot Rotation/1
  Real Position/2(RT) -> Robot Position/1
  Saturation/1 -> Divide2/2, Divide1/2  "WR"
  Divide/1 -> Sum1/2, Sum/2  "W*RR"
  Divide1/1 -> Right Wheel/1
  Divide2/1 -> Left Wheel/1
  Sum1/1 -> Divide1/1
  Sum/1 -> Divide2/1
  [W] -> Odometry/2(W)
  Odometry/1(RR) -> Odometry Rotation/1
  [V] -> Odometry/1(V)
  Odometry/2(RT) -> Odometry Position/1

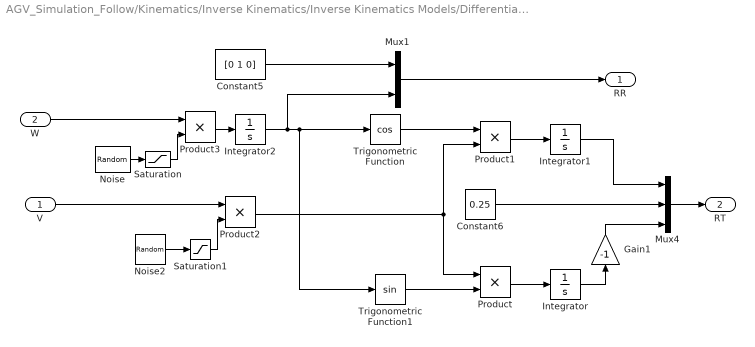
== system AGV_Simulation_Follow/Kinematics/Inverse Kinematics/Inverse Kinematics Models/Differential Drive Inverse Kinematics/Odometry ==
  V : Inport
  W : Inport  Port=2
  Constant5 : Constant  Value=[0 1 0]
  Constant6 : Constant  Value=0.25
  Gain1 : Gain  Gain=-1
  Integrator : Integrator  InitialCondition=InitPos(2)
  Integrator1 : Integrator  InitialCondition=InitPos(1)
  Integrator2 : Integrator  InitialCondition=InitRot
  Mux1 : Mux  Inputs=2
  Mux4 : Mux  Inputs=3
  Noise : RandomNumber  Mean=1  Variance=0.05  SampleTime=0.1
  Noise2 : RandomNumber  Mean=1  Variance=0.05  Seed=1  SampleTime=0.1
  Product{,1..3} (4 alike) : Product
  Saturation : Saturate  UpperLimit=1.2  LowerLimit=0.9
  Saturation1 : Saturate  UpperLimit=1.2  LowerLimit=0.9
  Trigonometric Function : Trigonometry  Operator=cos
  Trigonometric Function1 : Trigonometry
  RR : Outport
  RT : Outport  Port=2
  wires:
  Trigonometric Function1/1 -> Product/2
  Mux4/1 -> RT/1
  Product1/1 -> Integrator1/1
  Constant6/1 -> Mux4/2
  Trigonometric Function/1 -> Product1/1
  Product/1 -> Integrator/1
  Mux1/1 -> RR/1
  Product3/1 -> Integrator2/1
  Product2/1 -> Product/1, Product1/2
  Gain1/1 -> Mux4/3
  Integrator1/1 -> Mux4/1
  Integrator/1 -> Gain1/1
  Integrator2/1 -> Mux1/2, Trigonometric Function1/1, Trigonometric Function/1
  Constant5/1 -> Mux1/1
  V/1 -> Product2/1
  W/1 -> Product3/1
  Saturation/1 -> Product3/2
  Saturation1/1 -> Product2/2
  Noise2/1 -> Saturation1/1
  Noise/1 -> Saturation/1

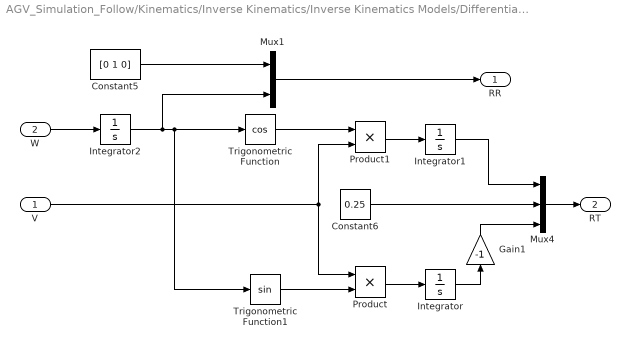
== system AGV_Simulation_Follow/Kinematics/Inverse Kinematics/Inverse Kinematics Models/Differential Drive Inverse Kinematics/Real Position ==
  V : Inport
  W : Inport  Port=2
  Constant5 : Constant  Value=[0 1 0]
  Constant6 : Constant  Value=0.25
  Gain1 : Gain  Gain=-1
  Integrator : Integrator  InitialCondition=InitPos(2)
  Integrator1 : Integrator  InitialCondition=InitPos(1)
  Integrator2 : Integrator  InitialCondition=InitRot
  Mux1 : Mux  Inputs=2
  Mux4 : Mux  Inputs=3
  Product : Product
  Product1 : Product
  Trigonometric Function : Trigonometry  Operator=cos
  Trigonometric Function1 : Trigonometry
  RR : Outport
  RT : Outport  Port=2
  wires:
  Trigonometric Function1/1 -> Product/2
  Mux4/1 -> RT/1
  Product1/1 -> Integrator1/1
  Constant6/1 -> Mux4/2
  Trigonometric Function/1 -> Product1/1
  Product/1 -> Integrator/1
  Mux1/1 -> RR/1
  W/1 -> Integrator2/1
  V/1 -> Product/1, Product1/2
  Gain1/1 -> Mux4/3
  Integrator1/1 -> Mux4/1
  Integrator/1 -> Gain1/1
  Integrator2/1 -> Mux1/2, Trigonometric Function1/1, Trigonometric Function/1
  Constant5/1 -> Mux1/1

== stateflow chart AGV_Simulation_Follow/Kinematics/Inverse Kinematics/Inverse Control Algorithms ==
  settings: executeAtInitialization=1
  state Control [parallel]
    settings: executionOrder=1
    state Differential_Drive
      state Initialize
        en:
        Thetasp=0;
        colision=0;
        stop_sim=0;
      state Go_linear
        en:
        Vx=1;
        W=0;
      state Start_sim
        en:
        Vx=0;
        W=0;
        colision=1;
      state Rotate_right
        en:
        Vx=0;
        Thetasp=Theta-pi/2;
        W=-pi/5;
      state Rotate_left
        en:
        Vx=0;
        Thetasp=Theta-pi/2;
        W=+pi/5;
      state Stop_sim
        en:
        Vx=0;
        W=0;
        stop_sim=1;
      state Rotate_left_or_rightSS
        en:
        Vx=0;
        Thetasp=Theta-pi/2;
        W=pi/5*(-1 + 2*randi([0,1]))
      state Turn_Stop
        en:
        Vx=1;
        W=0;
      Initialize -> Go_linear [order 1]
      Go_linear -> Start_sim [order 2] : [any(LIDAR(60:100)>0 & LIDAR(60:100)<0.5 )|| any(LIDAR(100:140)>0 & LIDAR(100:140)<0.75 ) || any(LIDAR(140:180)>0 & LIDAR(140:180)<0.5)]
      Start_sim -> Rotate_left [order 1] : [all(LIDAR(60:100)>0.85 | LIDAR(60:100)<0) && any(LIDAR(140:180)<2 & LIDAR(140:180)>0) ]
      Initialize -> Stop_sim [order 2] : [(diffx < 0.5 & diffx > -0.5) && (diffy < 0.5 & diffy > -0.5)  ]
      (default) -> Initialize
      Turn_Stop -> Initialize : [all(LIDAR(60:180)<0 | LIDAR(60:180)>0.75 )]
      Go_linear -> Stop_sim [order 1] : [(diffx < 0.5 & diffx > -0.5) && (diffy < 0.5 & diffy > -0.5)  ]
      Start_sim -> Rotate_left_or_rightSS [order 3] : [(all(LIDAR(140:180)>0.70 | LIDAR(140:180)<0)) && (all(LIDAR(60:100)>0.70| LIDAR(60:100)<0))]
      Start_sim -> Rotate_right [order 2] : [all(LIDAR(140:180)>0.85 | LIDAR(140:180)<0) && any(LIDAR(60:100)<2 & LIDAR(60:100)>0) ]
      Rotate_right -> Turn_Stop : [all(LIDAR(60:180)<0 | LIDAR(60:180)>0.75 ) && after(0.3,sec)]
      Rotate_left -> Turn_Stop : [all(LIDAR(60:180)<0 | LIDAR(60:180)>0.75 ) && after(0.3,sec)]
      Rotate_left_or_rightSS -> Turn_Stop : [all(LIDAR(60:180)<0 | LIDAR(60:180)>0.75 ) && after(0.3,sec)]
    (default) -> Differential_Drive
  data: X input; Z input; Theta input; Front_Sens input; Vx output; W output; Thetasp local; Right_Sens input; Left_Sens input; Back_Sens input; Model input; Kinematics input; diffx input; LIDAR input; rtime local; r local; colision output; diffy input; stop_sim output; targetdir input
  events: CLOCK input EITHER_EDGE_EVENT

== matlab function AGV_Simulation_Follow/Visualization/Subsystem2/Subsystem3/MATLAB Function2 ==
  data: Op1 input; Model output; Op2 input; Op3 input; Op4 input; Option input
function Model = Select_Model(Op1,Op2,Op3,Op4,Option)

switch Option
    case 1
Model = Op1;
    case 2
Model = Op2;
    case 3
Model = Op3;
    case 4
Model = Op4;
    otherwise
Model = Op1;
end

== matlab function AGV_Simulation_Follow/Visualization/Video Viewer/Image Processing/MATLAB Function ==
  data: Image input uint8 size=[480,640,3]; y output int16 size=[1,3]
function y = fcn(Image)
I=Image;
rr=0;
centers=[0,0];
[centers, rr] = imfindcircles(I,[10 100],'ObjectPolarity','dark','sensitivity',0.9);
if (size(centers)<1) ;centers=[0,0]; rr=[0]; end
y = int16([centers(1,1:2),rr(1)]);
